simulink model "ellipsoid_PI"  (R2025b)
settings: Solver=ode45  StartTime=0  StopTime=200  FixedStep=0.01  MaxStep=0.01  RelTol=1e-4  AbsTol=1e-4  EnableMultiTasking=on
values from neighbouring files (symbols this model uses):
  F_sat = 4e5    (= 400000)    [wecSimInputFile.m]
  simu = simulationClass()    [optimalGainCalcIrregular.m]    (also in optimalGainCalcRegular.m; wecSimInputFile.m)
undefined symbols (not defined in the file or in its folder): body, controller, pto
libraries: WECSim_Lib_Frames x1, WECSim_Lib_Body_Elements x1, WECSim_Lib_PTOs x1
settings Model: Creator=mlawson  LastModifiedBy=nova
settings SolverCC: ZeroCrossControl=DisableAll  AlgebraicLoopSolver=LineSearch  AutoInsertRateTranBlk=on
settings DataIOCC: SaveFormat=Array  SaveOutput=off  SaveTime=off  ReturnWorkspaceOutputs=off
settings OptimizationCC: BlockReduction=off  DefaultParameterBehavior=Inlined  BufferReuse=off  LifeSpan=inf  SimCompilerOptimization=on
settings DebuggingCC: MergeDetectMultiDrivingBlocksExec=none  SolverPrmCheckMsg=warning  UnconnectedInputMsg=warning  UnconnectedOutputMsg=warning  UnconnectedLineMsg=warning  AllowSymbolicDim=off  StateNameClashWarn=warning  SFUnexpectedBacktrackingDiag=warning  SFNoUnconditionalDefaultTransitionDiag=warning  ArithmeticOperatorsInVariantConditions=warning
settings HardwareCC: ProdBitPerPointer=32.0  ProdBitPerSizeT=32.0  ProdBitPerPtrDiffT=32.0  ProdLargestAtomicFloat=None  ProdIntDivRoundTo=Undefined  ProdEndianess=Unspecified  ProdWordSize=32.0  ProdHWDeviceType=32-bit Generic
settings ModelReferenceCC: EnableRefExpFcnMdlSchedulingChecks=on  PropagateSignalLabelsOutOfModel=off
settings SFSimCC: SimUseLocalCustomCode=off  CustomCodeUndefinedFunction=UseInterfaceOnly
settings RTWCC: RTWUseLocalCustomCode=off  GPUComputeCapability=3.5
settings CodeAppCC: StateflowObjectComments=on
settings GRTTargetCC: TargetLangStandard=C89/C90 (ANSI)
settings ConfigComp: CovMetricSettings=dw  CovSaveCumulativeToWorkspaceVar=on  CovSaveSingleToWorkspaceVar=on  CovExternalEMLEnable=off  CovSFcnEnable=off
settings SimscapeCC: SimscapeNormalizeSystem=off
settings ConfigurationSet: Description=SimMechanics 2G
settings ExplorerConfigSet: SimMechanicsOpenEditorOnUpdate=off  InternalSimMechanicsExplorerSettings="<ExplorerConfiguration><canonicalview>default</canonicalview><TilePanel><TileInfo><Tiles Columns=\"1\" Count=\"1\" Rows=\"1\"><Column Left=\"2\" Weight=\"1\"/><Column Left=\"1335\"/><Row Top=\"2\" Weight=\"1\"/><Row Top=\"911\"/><Tile Height=\"1\" Width=\"1\" X=\"0\" Y=\"0\"/></Tiles></TileInfo><SceneInfo><SceneViewer><BGColor><R>0.60000002384185791</R><G>0.60000002384185791</G><B>0.60000002384185791</B></BGColor><Camera><Position><X>365.37645888990272</X><Y>-369.82486814446582</Y><Z>359.64809521743916</Z></Position><Center><X>-6.7351450971904585</X><Y>2.2867358426280204</Y><Z>-12.463508769654169</Z></Center><Up><X>-0.40824829046386307</X><Y>0.40824829046386307</Y><Z>0.81649658092772615</Z></Up><Left>-57.820127362122818</Left><Right>57.820127362122818</Right><Bottom>-38.308817187253304</Bottom><Top>38.308817187253304</Top></Camera></SceneViewer></SceneInfo></TilePanel></ExplorerConfiguration>"

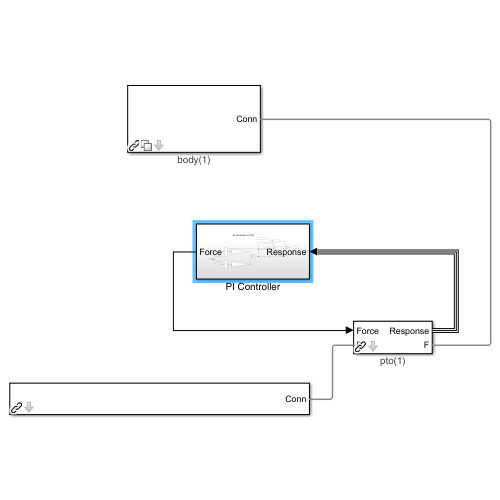
[thumbnail: Simulink's stored preview of the top-level diagram]
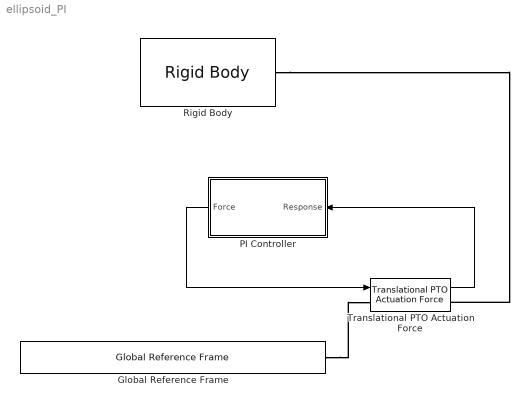
== system ellipsoid_PI ==
  Global Reference Frame : WECSim_Lib_Frames/Global Reference Frame  waves=waves  simu=simu
  PI Controller : Subsystem
  Rigid Body : WECSim_Lib_Body_Elements/Rigid Body  body=body(1)
  Translational PTO Actuation Force : WECSim_Lib_PTOs/Translational PTO Actuation Force  pto=pto(1)
      settings: AttributesFormatString=%<pto>
  wires:
  PI Controller/1(Force) -> Translational PTO Actuation Force/1
  Translational PTO Actuation Force/1 -> PI Controller/1(Response)
  connections:
  Global Reference Frame/RConn1 -- Translational PTO Actuation Force/LConn1
  Rigid Body/RConn1 -- Translational PTO Actuation Force/RConn1

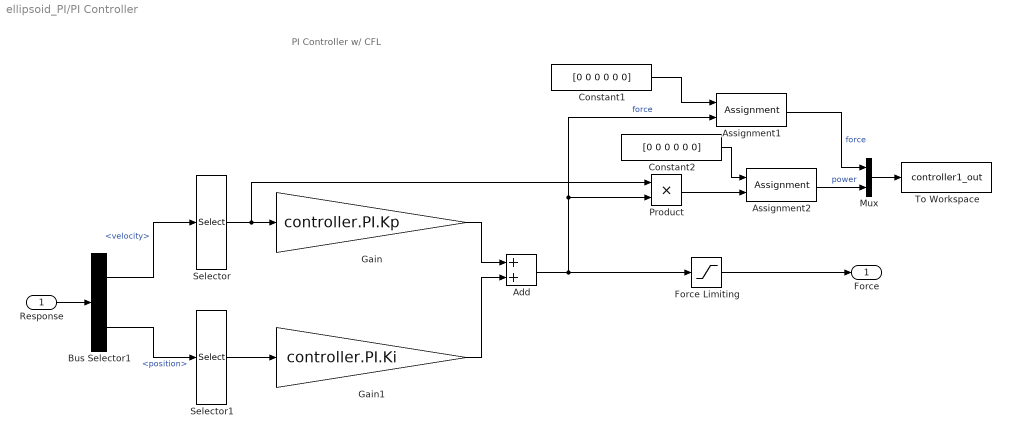
== system ellipsoid_PI/PI Controller ==
  note: PI Controller w/ CFL
  Response : Inport
  Add : Sum
  Assignment1 : Assignment  IndexOptions=Index vector (dialog)  Indices=3  OutputSizes=1
  Assignment2 : Assignment  IndexOptions=Index vector (dialog)  Indices=3  OutputSizes=1
  Bus Selector1 : BusSelector  OutputSignals=velocity,position
  Constant1 : Constant  Value=[0 0 0 0 0 0]
  Constant2 : Constant  Value=[0 0 0 0 0 0]
  Force Limiting : Saturate  UpperLimit=F_sat  LowerLimit=-F_sat
  Gain : Gain  Gain=controller.PI.Kp
  Gain1 : Gain  Gain=controller.PI.Ki
  Mux : Mux  Inputs=2
  Product : Product
  Selector : Selector  InputPortWidth=6  IndexOptions=Index vector (dialog)  Indices=3  OutputSizes=1
  Selector1 : Selector  InputPortWidth=6  IndexOptions=Index vector (dialog)  Indices=3  OutputSizes=1
  To Workspace : ToWorkspace  VariableName=controller1_out  SaveFormat=Structure With Time  SampleTime=simu.dtOut
  Force : Outport
  wires:
  Response/1 -> Bus Selector1/1
  Bus Selector1/2 -> Selector1/1  "<position>"
  Bus Selector1/1 -> Selector/1  "<velocity>"
  Selector/1 -> Product/1, Gain/1
  Selector1/1 -> Gain1/1
  Gain/1 -> Add/1
  Gain1/1 -> Add/2
  Add/1 -> Product/2, Assignment1/2, Force Limiting/1  "force"
  Mux/1 -> To Workspace/1
  Constant2/1 -> Assignment2/1
  Product/1 -> Assignment2/2
  Constant1/1 -> Assignment1/1
  Assignment1/1 -> Mux/1  "force"
  Assignment2/1 -> Mux/2  "power"
  Force Limiting/1 -> Force/1
